simulink model "test_chamber_block"  (R2024b)
settings: Solver=FixedStepDiscrete  StartTime=0.0  StopTime=8  FixedStep=1e-3  RelTol=1e-3
settings Model: Creator=sammy  LastModifiedBy=sammy

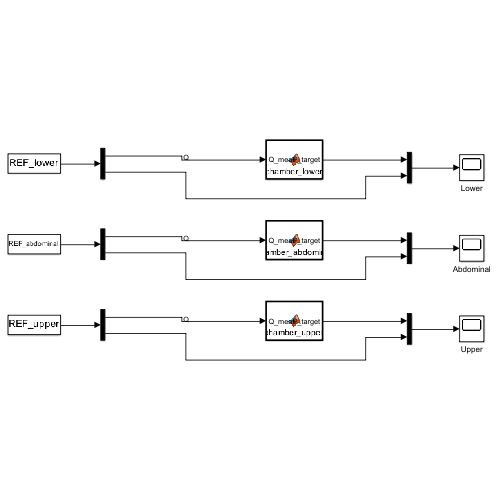
[thumbnail: Simulink's stored preview of the top-level diagram]
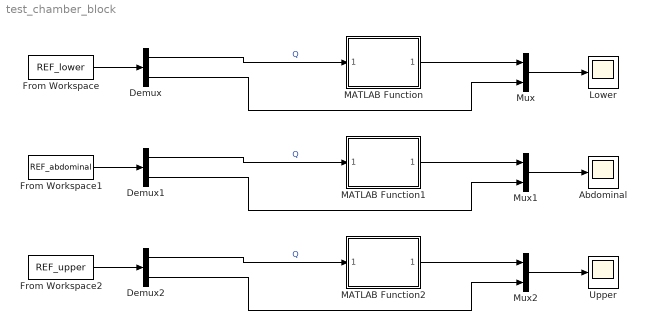
== system test_chamber_block ==
  Abdominal : Scope
  Demux : Demux  Outputs=2
  Demux1 : Demux  Outputs=2
  Demux2 : Demux  Outputs=2
  From Workspace : FromWorkspace  VariableName=REF_lower  SampleTime=1e-3  OutputAfterFinalValue=Holding final value
  From Workspace1 : FromWorkspace  VariableName=REF_abdominal  SampleTime=1e-3  OutputAfterFinalValue=Holding final value
  From Workspace2 : FromWorkspace  VariableName=REF_upper  SampleTime=1e-3  OutputAfterFinalValue=Holding final value
  Lower : Scope
  MATLAB Function : MATLAB Function  TreatAsAtomicUnit=on
  MATLAB Function1 : MATLAB Function  TreatAsAtomicUnit=on
  MATLAB Function2 : MATLAB Function  TreatAsAtomicUnit=on
  Mux : Mux  Inputs=2
  Mux1 : Mux  Inputs=2
  Mux2 : Mux  Inputs=2
  Upper : Scope
  wires:
  From Workspace/1 -> Demux/1
  Demux/1 -> MATLAB Function/1(Q_meas)  "Q"
  Demux/2 -> Mux/2
  MATLAB Function/1(P_target) -> Mux/1
  Mux/1 -> Lower/1
  Demux1/2 -> Mux1/2
  MATLAB Function1/1(P_target) -> Mux1/1
  Demux1/1 -> MATLAB Function1/1(Q_meas)  "Q"
  Mux1/1 -> Abdominal/1
  From Workspace1/1 -> Demux1/1
  From Workspace2/1 -> Demux2/1
  MATLAB Function2/1(P_target) -> Mux2/1
  Demux2/2 -> Mux2/2
  Mux2/1 -> Upper/1
  Demux2/1 -> MATLAB Function2/1(Q_meas)  "Q"

== matlab function test_chamber_block/MATLAB Function ==
  data: Q_meas input; P_target output; S_lower parameter
   function P_target = chamber_lower(Q_meas, S_lower)
   %#codegen
   persistent A Q Pn Pc
   S = S_lower;
   if isempty(A)
       A  = S.A0;  Q = zeros(S.nF,1);
       Pn = S.Pref*ones(S.nNodes,1);  Pc = S.Pref*ones(numel(S.tSeg),1);
   end
   [A, Q, Pn, Pc] = charlton1d_step(S, A, Q, Pn, Pc, 1e-6*Q_meas);
   P_target = Pn(S.root)/133.322;

== matlab function test_chamber_block/MATLAB Function2 ==
  data: Q_meas input; P_target output; S_upper parameter
function P_target = chamber_upper(Q_meas, S_upper)
   %#codegen
   persistent A Q Pn Pc
   S = S_upper;
   if isempty(A)
       A  = S.A0;  Q = zeros(S.nF,1);
       Pn = S.Pref*ones(S.nNodes,1);  Pc = S.Pref*ones(numel(S.tSeg),1);
   end
   [A, Q, Pn, Pc] = charlton1d_step(S, A, Q, Pn, Pc, 1e-6*Q_meas);
   P_target = Pn(S.root)/133.322;

== matlab function test_chamber_block/MATLAB Function1 ==
  data: Q_meas input; P_target output; S_abdominal parameter
function P_target = chamber_abdominal(Q_meas, S_abdominal)
   %#codegen
   persistent A Q Pn Pc
   S = S_abdominal;
   if isempty(A)
       A  = S.A0;  Q = zeros(S.nF,1);
       Pn = S.Pref*ones(S.nNodes,1);  Pc = S.Pref*ones(numel(S.tSeg),1);
   end
   [A, Q, Pn, Pc] = charlton1d_step(S, A, Q, Pn, Pc, 1e-6*Q_meas);
   P_target = Pn(S.root)/133.322;
